simulink model "modele_chaine_complete_codee"  (R2024b)
settings: Solver=FixedStepDiscrete  StartTime=0.0  StopTime=(Nsim-1)*Tb  FixedStep=Tpas  RelTol=1e-3
values from neighbouring files (symbols this model uses):
  L = @(a, b) add_line(blk, a, b, 'autorouting', 'on')    [ajouter_codeur_registre.m]    (also in ajouter_decodeur_hamming.m; ajouter_modem_qpsk.m; ajouter_modem_qpsk_filtre.m; construire_modele_codeur_registre.m = @(a, b) add_line(mdl, a, b, 'autorouting', 'on'))
undefined symbols (not defined in the file or in its folder): dAlign, dPhase, graine, hc, hE, N0, phaseC, Tb, Tc, Te
settings Model: Creator=youka  LastModifiedBy=youka

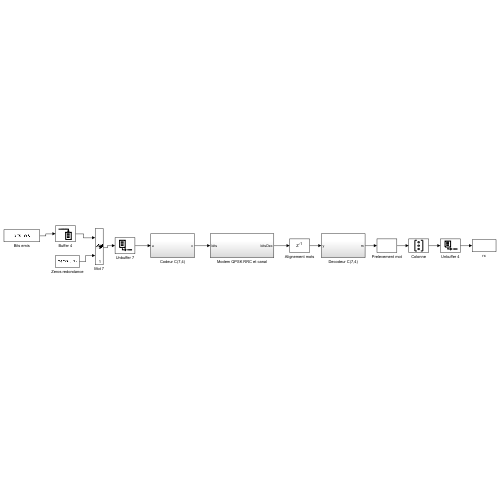
[thumbnail: Simulink's stored preview of the top-level diagram]
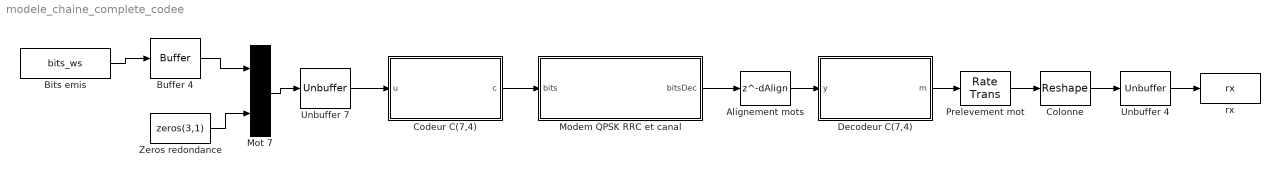
== system modele_chaine_complete_codee ==
  Alignement mots : Delay  DelayLength=dAlign
  Bits emis : FromWorkspace  VariableName=bits_ws  SampleTime=Tb  Interpolate=off  OutputAfterFinalValue=Setting to zero
  Buffer 4 : Buffer  N=4
  Codeur C(7,4) : Subsystem
  Colonne : Reshape  OutputDimensionality=Column vector (2-D)
  Decodeur C(7,4) : Subsystem
  Modem QPSK RRC et canal : Subsystem
  Mot 7 : Concatenate  Mode=Multidimensional array
  Prelevement mot : RateTransition  OutPortSampleTime=4*Tb
  Unbuffer 4 : Unbuffer
  Unbuffer 7 : Unbuffer
  Zeros redondance : Constant  Value=zeros(3,1)  SampleTime=4*Tb
  rx : ToWorkspace  VariableName=rx  SampleTime=-1
  wires:
  Bits emis/1 -> Buffer 4/1
  Buffer 4/1 -> Mot 7/1
  Zeros redondance/1 -> Mot 7/2
  Mot 7/1 -> Unbuffer 7/1
  Unbuffer 7/1 -> Codeur C(7,4)/1(u)
  Codeur C(7,4)/1(c) -> Modem QPSK RRC et canal/1(bits)
  Modem QPSK RRC et canal/1(bitsDec) -> Alignement mots/1
  Alignement mots/1 -> Decodeur C(7,4)/1(y)
  Decodeur C(7,4)/1(m) -> Prelevement mot/1
  Prelevement mot/1 -> Colonne/1
  Colonne/1 -> Unbuffer 4/1
  Unbuffer 4/1 -> rx/1

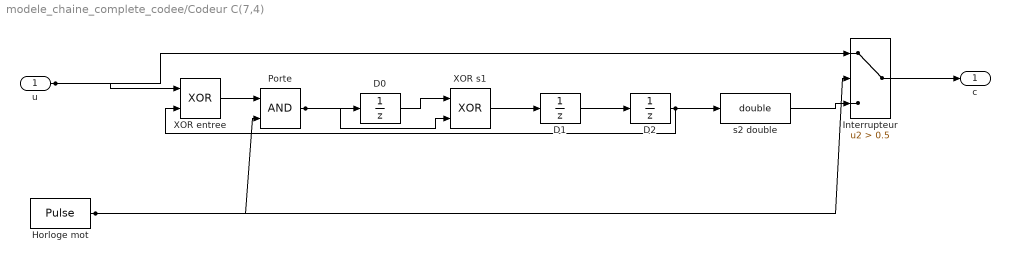
== system modele_chaine_complete_codee/Codeur C(7,4) ==
  u : Inport
  D0 : UnitDelay  SampleTime=Tc  HasFrameUpgradeWarning=on
  D1 : UnitDelay  SampleTime=Tc  HasFrameUpgradeWarning=on
  D2 : UnitDelay  SampleTime=Tc  HasFrameUpgradeWarning=on
  Horloge mot : DiscretePulseGenerator  Period=7  PulseWidth=4  PhaseDelay=phaseC  SampleTime=Tc
  Interrupteur : Switch  Criteria=u2 > Threshold  Threshold=0.5  SaturateOnIntegerOverflow=off  InputSameDT=off
  Porte : Logic  AllPortsSameDT=off  OutDataTypeStr=boolean
  XOR entree : Logic  Operator=XOR  AllPortsSameDT=off  OutDataTypeStr=boolean
  XOR s1 : Logic  Operator=XOR  AllPortsSameDT=off  OutDataTypeStr=boolean
  s2 double : DataTypeConversion  OutDataTypeStr=double  SaturateOnIntegerOverflow=off  RndMeth=Floor
  c : Outport
  wires:
  u/1 -> XOR entree/1, Interrupteur/1
  D2/1 -> XOR entree/2, s2 double/1
  XOR entree/1 -> Porte/1
  Horloge mot/1 -> Porte/2, Interrupteur/2
  Porte/1 -> D0/1, XOR s1/2
  D0/1 -> XOR s1/1
  XOR s1/1 -> D1/1
  D1/1 -> D2/1
  s2 double/1 -> Interrupteur/3
  Interrupteur/1 -> c/1

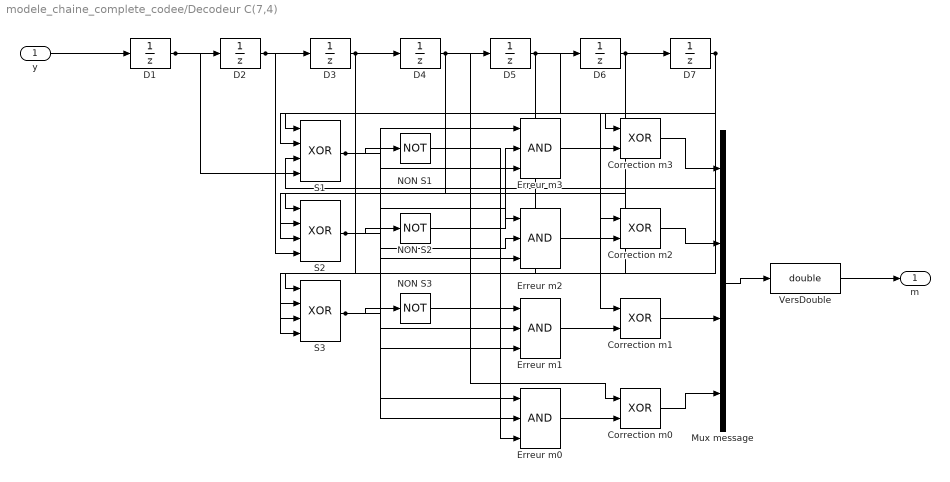
== system modele_chaine_complete_codee/Decodeur C(7,4) ==
  y : Inport
  Correction m{0..3} (4 alike) : Logic  Operator=XOR  AllPortsSameDT=off  OutDataTypeStr=boolean
  D{1..7} (7 alike) : UnitDelay  SampleTime=Tc  HasFrameUpgradeWarning=on
  Erreur m{0..3} (4 alike) : Logic  Inputs=3  AllPortsSameDT=off  OutDataTypeStr=boolean
  Mux message : Mux
  NON S1 : Logic  Operator=NOT  AllPortsSameDT=off  OutDataTypeStr=boolean
  NON S2 : Logic  Operator=NOT  AllPortsSameDT=off  OutDataTypeStr=boolean
  NON S3 : Logic  Operator=NOT  AllPortsSameDT=off  OutDataTypeStr=boolean
  S1 : Logic  Operator=XOR  Inputs=4  AllPortsSameDT=off  OutDataTypeStr=boolean
  S2 : Logic  Operator=XOR  Inputs=4  AllPortsSameDT=off  OutDataTypeStr=boolean
  S3 : Logic  Operator=XOR  Inputs=4  AllPortsSameDT=off  OutDataTypeStr=boolean
  VersDouble : DataTypeConversion  OutDataTypeStr=double  SaturateOnIntegerOverflow=off  RndMeth=Floor
  m : Outport
  wires:
  y/1 -> D1/1
  D1/1 -> D2/1, S1/4
  D2/1 -> D3/1, S2/4
  D3/1 -> D4/1, S3/4
  D4/1 -> D5/1, S1/1, S2/1, Correction m0/1
  D5/1 -> D6/1, S2/2, S3/1, Correction m1/1
  D6/1 -> D7/1, S1/2, S2/3, S3/2, Correction m2/1
  D7/1 -> S1/3, S3/3, Correction m3/1
  S1/1 -> NON S1/1, Erreur m3/1, Erreur m2/1, Erreur m0/1
  S2/1 -> NON S2/1, Erreur m2/2, Erreur m1/2, Erreur m0/2
  S3/1 -> NON S3/1, Erreur m3/3, Erreur m2/3, Erreur m1/3
  NON S2/1 -> Erreur m3/2
  Erreur m3/1 -> Correction m3/2
  Erreur m2/1 -> Correction m2/2
  NON S1/1 -> Erreur m1/1
  Erreur m1/1 -> Correction m1/2
  NON S3/1 -> Erreur m0/3
  Erreur m0/1 -> Correction m0/2
  Correction m3/1 -> Mux message/1
  Correction m2/1 -> Mux message/2
  Correction m1/1 -> Mux message/3
  Correction m0/1 -> Mux message/4
  Mux message/1 -> VersDouble/1
  VersDouble/1 -> m/1

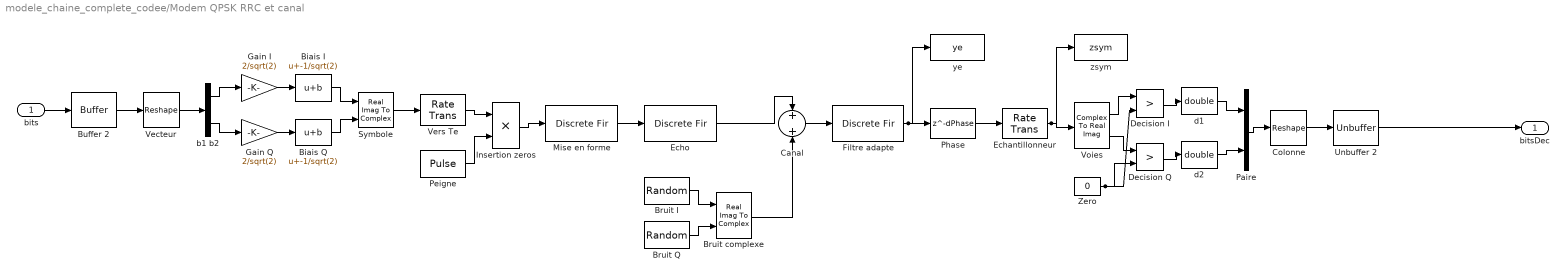
== system modele_chaine_complete_codee/Modem QPSK RRC et canal ==
  bits : Inport
  Biais I : Bias  Bias=-1/sqrt(2)  SaturateOnIntegerOverflow=off
  Biais Q : Bias  Bias=-1/sqrt(2)  SaturateOnIntegerOverflow=off
  Bruit I : RandomNumber  Variance=N0/2  Seed=graine+1  SampleTime=Te
  Bruit Q : RandomNumber  Variance=N0/2  Seed=graine+2  SampleTime=Te
  Bruit complexe : RealImagToComplex
  Buffer 2 : Buffer  N=2
  Canal : Sum
  Colonne : Reshape  OutputDimensionality=Column vector (2-D)
  Decision I : RelationalOperator  Operator=>  OutDataTypeStr=boolean  RndMeth=Simplest  InputSameDT=off
  Decision Q : RelationalOperator  Operator=>  OutDataTypeStr=boolean  RndMeth=Simplest  InputSameDT=off
  Echantillonneur : RateTransition  OutPortSampleTime=Tsym
  Echo : DiscreteFir  Coefficients=hc
  Filtre adapte : DiscreteFir  Coefficients=fliplr(hE)
  Gain I : Gain  Gain=2/sqrt(2)
  Gain Q : Gain  Gain=2/sqrt(2)
  Insertion zeros : Product  Inputs=**
  Mise en forme : DiscreteFir  Coefficients=hE
  Paire : Mux  Inputs=2
  Peigne : DiscretePulseGenerator  Period=L  SampleTime=Te
  Phase : Delay  DelayLength=dPhase
  Symbole : RealImagToComplex
  Unbuffer 2 : Unbuffer
  Vecteur : Reshape
  Vers Te : RateTransition  OutPortSampleTime=Te
  Voies : ComplexToRealImag
  Zero : Constant  Value=0
  b1 b2 : Demux  Outputs=2
  d1 : DataTypeConversion  OutDataTypeStr=double  SaturateOnIntegerOverflow=off  RndMeth=Floor
  d2 : DataTypeConversion  OutDataTypeStr=double  SaturateOnIntegerOverflow=off  RndMeth=Floor
  ye : ToWorkspace  VariableName=ye  SampleTime=-1
      settings: MaxDataPoints=Nlog
  zsym : ToWorkspace  VariableName=zsym  SampleTime=-1
  bitsDec : Outport
  wires:
  bits/1 -> Buffer 2/1
  Buffer 2/1 -> Vecteur/1
  Vecteur/1 -> b1 b2/1
  b1 b2/1 -> Gain I/1
  Gain I/1 -> Biais I/1
  Biais I/1 -> Symbole/1
  b1 b2/2 -> Gain Q/1
  Gain Q/1 -> Biais Q/1
  Biais Q/1 -> Symbole/2
  Symbole/1 -> Vers Te/1
  Vers Te/1 -> Insertion zeros/1
  Peigne/1 -> Insertion zeros/2
  Insertion zeros/1 -> Mise en forme/1
  Mise en forme/1 -> Echo/1
  Bruit I/1 -> Bruit complexe/1
  Bruit Q/1 -> Bruit complexe/2
  Echo/1 -> Canal/1
  Bruit complexe/1 -> Canal/2
  Canal/1 -> Filtre adapte/1
  Filtre adapte/1 -> ye/1, Phase/1
  Phase/1 -> Echantillonneur/1
  Echantillonneur/1 -> zsym/1, Voies/1
  Voies/1 -> Decision I/1
  Zero/1 -> Decision I/2, Decision Q/2
  Voies/2 -> Decision Q/1
  Decision I/1 -> d1/1
  Decision Q/1 -> d2/1
  d1/1 -> Paire/1
  d2/1 -> Paire/2
  Paire/1 -> Colonne/1
  Colonne/1 -> Unbuffer 2/1
  Unbuffer 2/1 -> bitsDec/1
